simulink model "BMS_CC_CV_79kW"  (R2026a)
settings: Solver=FixedStepDiscrete  StopTime=3600  FixedStep=1
undefined symbols (not defined in the file or in its folder): DiscIntNeverNeededParam
libraries: simulink x8
settings Model: Creator=anish  LastModifiedBy=anish

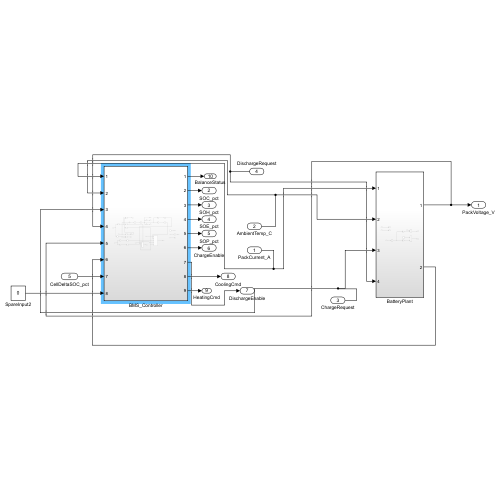
[thumbnail: Simulink's stored preview of the top-level diagram]
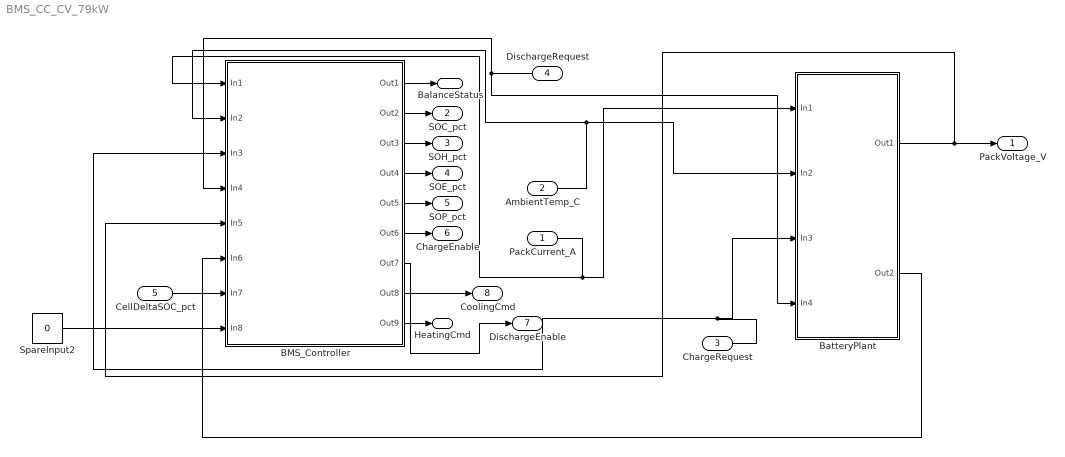
== system BMS_CC_CV_79kW ==
  PackCurrent_A : Inport  OutDataTypeStr=double
  AmbientTemp_C : Inport  Port=2  OutDataTypeStr=double
  ChargeRequest : Inport  Port=3  OutDataTypeStr=double
  DischargeRequest : Inport  Port=4  OutDataTypeStr=double
  CellDeltaSOC_pct : Inport  Port=5  OutDataTypeStr=double
  BMS_Controller : Subsystem
  BatteryPlant : Subsystem
  SpareInput2 : Constant  Value=0
  PackVoltage_V : Outport
  SOC_pct : Outport  Port=2
  SOH_pct : Outport  Port=3
  SOE_pct : Outport  Port=4
  SOP_pct : Outport  Port=5
  ChargeEnable : Outport  Port=6
  DischargeEnable : Outport  Port=7
  CoolingCmd : Outport  Port=8
  HeatingCmd : Outport  Port=9
  BalanceStatus : Outport  Port=10
  wires:
  PackCurrent_A/1 -> BatteryPlant/1(In1), BMS_Controller/1(In1)
  AmbientTemp_C/1 -> BMS_Controller/2(In2), BatteryPlant/2(In2)
  ChargeRequest/1 -> BatteryPlant/3(In3), BMS_Controller/3(In3)
  DischargeRequest/1 -> BMS_Controller/4(In4), BatteryPlant/4(In4)
  BatteryPlant/1(Out1) -> BMS_Controller/5(In5), PackVoltage_V/1
  BatteryPlant/2(Out2) -> BMS_Controller/6(In6)
  SpareInput2/1 -> BMS_Controller/8(In8)
  BMS_Controller/2(Out2) -> SOC_pct/1
  BMS_Controller/3(Out3) -> SOH_pct/1
  BMS_Controller/4(Out4) -> SOE_pct/1
  BMS_Controller/5(Out5) -> SOP_pct/1
  BMS_Controller/6(Out6) -> ChargeEnable/1
  BMS_Controller/7(Out7) -> DischargeEnable/1
  BMS_Controller/8(Out8) -> CoolingCmd/1
  BMS_Controller/9(Out9) -> HeatingCmd/1
  BMS_Controller/1(Out1) -> BalanceStatus/1
  CellDeltaSOC_pct/1 -> BMS_Controller/7(In7)

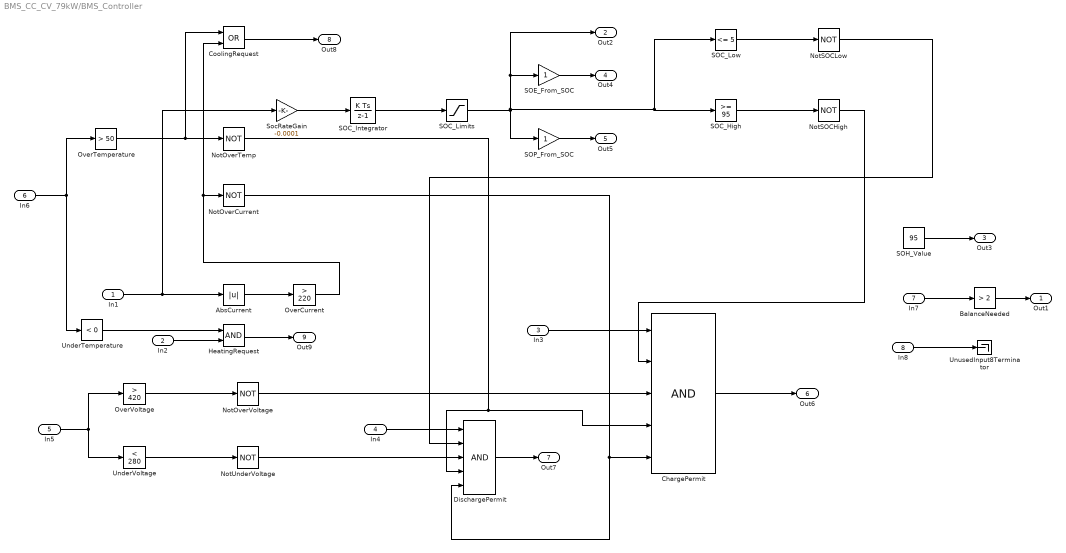
== system BMS_CC_CV_79kW/BMS_Controller ==
  In1 : Inport  OutDataTypeStr=double
  In2 : Inport  Port=2  OutDataTypeStr=double
  In3 : Inport  Port=3  OutDataTypeStr=double
  In4 : Inport  Port=4  OutDataTypeStr=double
  In5 : Inport  Port=5  OutDataTypeStr=double
  In6 : Inport  Port=6  OutDataTypeStr=double
  In7 : Inport  Port=7  OutDataTypeStr=double
  In8 : Inport  Port=8  OutDataTypeStr=double
  AbsCurrent : Abs  SaturateOnIntegerOverflow=off
  BalanceNeeded : simulink/Logic and Bit Operations/Compare To Constant  relop=>  const=2  OutDataTypeStr=boolean
  ChargePermit : Logic  Inputs=5  AllPortsSameDT=off  OutDataTypeStr=boolean
  CoolingRequest : Logic  Operator=OR  AllPortsSameDT=off  OutDataTypeStr=boolean
  DischargePermit : Logic  Inputs=5  AllPortsSameDT=off  OutDataTypeStr=boolean
  HeatingRequest : Logic  AllPortsSameDT=off  OutDataTypeStr=boolean
  NotOverCurrent : Logic  Operator=NOT  AllPortsSameDT=off  OutDataTypeStr=boolean
  NotOverTemp : Logic  Operator=NOT  AllPortsSameDT=off  OutDataTypeStr=boolean
  NotOverVoltage : Logic  Operator=NOT  AllPortsSameDT=off  OutDataTypeStr=boolean
  NotSOCHigh : Logic  Operator=NOT  AllPortsSameDT=off  OutDataTypeStr=boolean
  NotSOCLow : Logic  Operator=NOT  AllPortsSameDT=off  OutDataTypeStr=boolean
  NotUnderVoltage : Logic  Operator=NOT  AllPortsSameDT=off  OutDataTypeStr=boolean
  OverCurrent : simulink/Logic and Bit Operations/Compare To Constant  relop=>  const=220  OutDataTypeStr=boolean
  OverTemperature : simulink/Logic and Bit Operations/Compare To Constant  relop=>  const=50  OutDataTypeStr=boolean
  OverVoltage : simulink/Logic and Bit Operations/Compare To Constant  relop=>  const=420  OutDataTypeStr=boolean
  SOC_High : simulink/Logic and Bit Operations/Compare To Constant  relop=>=  const=95  OutDataTypeStr=boolean
  SOC_Integrator : DiscreteIntegrator  InitialCondition=80  ICPrevOutput=DiscIntNeverNeededParam  ICPrevScaledInput=DiscIntNeverNeededParam
  SOC_Limits : Saturate  UpperLimit=100  LowerLimit=0
  SOC_Low : simulink/Logic and Bit Operations/Compare To Constant  relop=<=  const=5  OutDataTypeStr=boolean
  SOE_From_SOC : Gain
  SOH_Value : Constant  Value=95
  SOP_From_SOC : Gain
  SocRateGain : Gain  Gain=-0.0001
  UnderTemperature : simulink/Logic and Bit Operations/Compare To Constant  relop=<  const=0  OutDataTypeStr=boolean
  UnderVoltage : simulink/Logic and Bit Operations/Compare To Constant  relop=<  const=280  OutDataTypeStr=boolean
  UnusedInput8Terminator : Terminator
  Out1 : Outport
  Out2 : Outport  Port=2
  Out3 : Outport  Port=3
  Out4 : Outport  Port=4
  Out5 : Outport  Port=5
  Out6 : Outport  Port=6
  Out7 : Outport  Port=7
  Out8 : Outport  Port=8
  Out9 : Outport  Port=9
  wires:
  In1/1 -> SocRateGain/1, AbsCurrent/1
  SocRateGain/1 -> SOC_Integrator/1
  SOC_Integrator/1 -> SOC_Limits/1
  SOC_Limits/1 -> Out2/1, SOE_From_SOC/1, SOC_Low/1, SOC_High/1, SOP_From_SOC/1
  SOE_From_SOC/1 -> Out4/1
  SOP_From_SOC/1 -> Out5/1
  SOH_Value/1 -> Out3/1
  In5/1 -> OverVoltage/1, UnderVoltage/1
  In6/1 -> OverTemperature/1, UnderTemperature/1
  AbsCurrent/1 -> OverCurrent/1
  SOC_High/1 -> NotSOCHigh/1
  SOC_Low/1 -> NotSOCLow/1
  OverVoltage/1 -> NotOverVoltage/1
  UnderVoltage/1 -> NotUnderVoltage/1
  OverTemperature/1 -> NotOverTemp/1, CoolingRequest/1
  OverCurrent/1 -> CoolingRequest/2, NotOverCurrent/1
  In3/1 -> ChargePermit/1
  NotSOCHigh/1 -> ChargePermit/2
  NotOverVoltage/1 -> ChargePermit/3
  NotOverTemp/1 -> ChargePermit/4, DischargePermit/4
  ChargePermit/1 -> Out6/1
  In4/1 -> DischargePermit/1
  NotSOCLow/1 -> DischargePermit/2
  NotUnderVoltage/1 -> DischargePermit/3
  DischargePermit/1 -> Out7/1
  CoolingRequest/1 -> Out8/1
  UnderTemperature/1 -> HeatingRequest/1
  In2/1 -> HeatingRequest/2
  HeatingRequest/1 -> Out9/1
  In8/1 -> UnusedInput8Terminator/1
  NotOverCurrent/1 -> ChargePermit/5, DischargePermit/5
  In7/1 -> BalanceNeeded/1
  BalanceNeeded/1 -> Out1/1

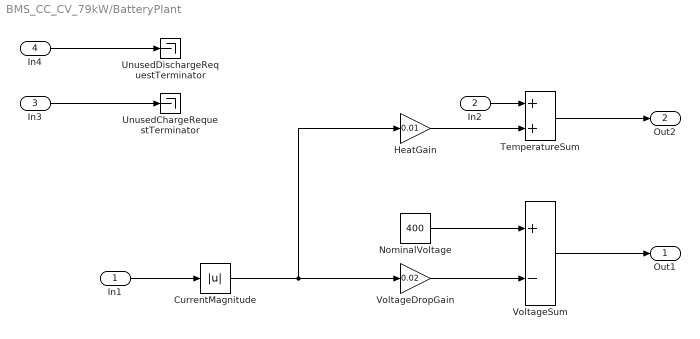
== system BMS_CC_CV_79kW/BatteryPlant ==
  In1 : Inport
  In2 : Inport  Port=2
  In3 : Inport  Port=3
  In4 : Inport  Port=4
  CurrentMagnitude : Abs  SaturateOnIntegerOverflow=off
  HeatGain : Gain  Gain=0.01
  NominalVoltage : Constant  Value=400
  TemperatureSum : Sum
  UnusedChargeRequestTerminator : Terminator
  UnusedDischargeRequestTerminator : Terminator
  VoltageDropGain : Gain  Gain=0.02
  VoltageSum : Sum  Inputs=+-
  Out1 : Outport  OutDataTypeStr=double
  Out2 : Outport  Port=2  OutDataTypeStr=double
  wires:
  In1/1 -> CurrentMagnitude/1
  CurrentMagnitude/1 -> VoltageDropGain/1, HeatGain/1
  NominalVoltage/1 -> VoltageSum/1
  VoltageDropGain/1 -> VoltageSum/2
  VoltageSum/1 -> Out1/1
  In2/1 -> TemperatureSum/1
  HeatGain/1 -> TemperatureSum/2
  TemperatureSum/1 -> Out2/1
  In3/1 -> UnusedChargeRequestTerminator/1
  In4/1 -> UnusedDischargeRequestTerminator/1
